simulink model "stall_detection_block_v2"  (R2022b)
settings: Solver=FixedStepAuto  StartTime=0.0  StopTime=inf  FixedStep=0.002  RelTol=1e-3  EnableMultiTasking=on
undefined symbols (not defined in the file or in its folder): DiscIntNeverNeededParam
libraries: quarc_library x1
settings Model: Creator=christopher.oneill  LastModifiedBy=christopher.oneill
settings SolverCC: PositivePriorityOrder=on
settings RTWCC: Description=QUARC Win64 Target Using Toolchain  SystemTargetFile=quarc_win64.tlc  Toolchain=QUARC win64 | nmake (64-bit Windows)  BuildConfiguration=Faster Runs
settings STFCustomTargetCC: TargetLangStandard=C99 (ISO)  ConcurrentExecutionCompliant=on  GRTInterface=on  UseToolchainInfoCompliant=on  SystemTargetFile=quarc_win64.tlc
settings GRTTargetCC: ParMdlRefBuildCompliant=off  CompOptLevelCompliant=off  CombineOutputUpdateFcns=off  MatFileLogging=off  CPPClassGenCompliant=off  GRTInterface=on  ExtMode=on  ExtModeMexFile=quarc_comm

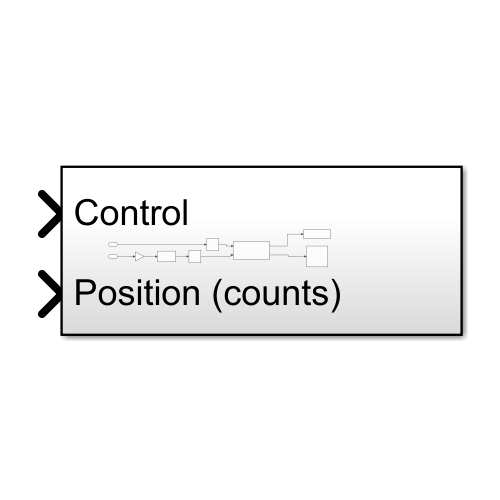
[thumbnail: Simulink's stored preview of the top-level diagram]
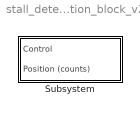
== system stall_detection_block_v2 ==
  Subsystem : Subsystem

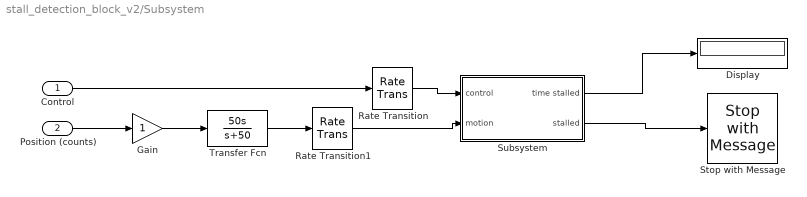
== system stall_detection_block_v2/Subsystem ==
  Control : Inport
  Position (counts) : Inport  Port=2
  Display : Display
  Gain : Gain
  Rate Transition : RateTransition
  Rate Transition1 : RateTransition
  Stop with Message : quarc_library/Sinks/Error Handling/Stop with Message  message_type=Fixed error message  message_icon=Error  message=Stall Detected! Please snsure that the DC motor is free to move and is functioning properly. Please ask a TA to check your code if you have recived this error.
  Subsystem : Subsystem
  Transfer Fcn : TransferFcn  Numerator=[50 0]  Denominator=[1 50]
  wires:
  Control/1 -> Rate Transition/1
  Position (counts)/1 -> Gain/1
  Gain/1 -> Transfer Fcn/1
  Transfer Fcn/1 -> Rate Transition1/1
  Rate Transition1/1 -> Subsystem/2(motion)
  Rate Transition/1 -> Subsystem/1(control)
  Subsystem/1(time stalled) -> Display/1
  Subsystem/2(stalled) -> Stop with Message/1

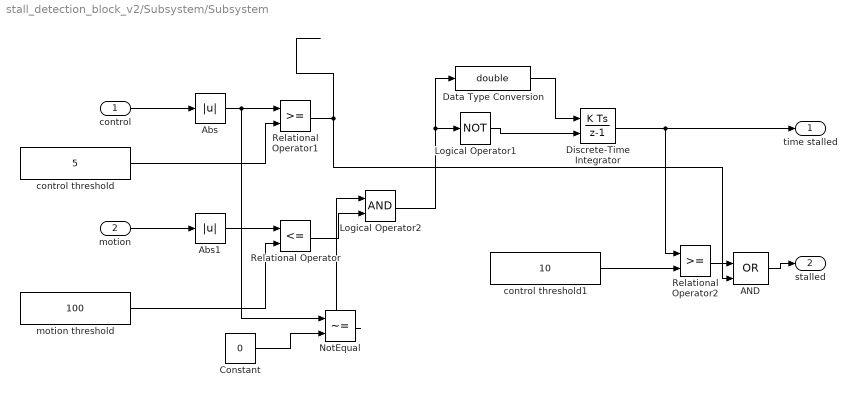
== system stall_detection_block_v2/Subsystem/Subsystem ==
  control : Inport
  motion : Inport  Port=2
  AND : Logic  Operator=OR  IconShape=distinctive  AllPortsSameDT=off  OutDataTypeStr=boolean
  Abs : Abs  SaturateOnIntegerOverflow=off
  Abs1 : Abs  SaturateOnIntegerOverflow=off
  Constant : Constant  Value=0
  Data Type Conversion : DataTypeConversion  OutDataTypeStr=double  SaturateOnIntegerOverflow=off  RndMeth=Floor
  Discrete-Time Integrator : DiscreteIntegrator  ExternalReset=rising  InitialConditionSetting=Compatibility  SampleTime=-1  ICPrevOutput=DiscIntNeverNeededParam  ICPrevScaledInput=DiscIntNeverNeededParam
  Logical Operator1 : Logic  Operator=NOT  AllPortsSameDT=off  OutDataTypeStr=boolean
  Logical Operator2 : Logic  AllPortsSameDT=off  OutDataTypeStr=boolean
  NotEqual : RelationalOperator  Operator=~=  OutDataTypeStr=boolean  RndMeth=Simplest  InputSameDT=off
  Relational Operator : RelationalOperator  Operator=<=  OutDataTypeStr=boolean  InputSameDT=off
  Relational Operator1 : RelationalOperator  OutDataTypeStr=boolean  InputSameDT=off
  Relational Operator2 : RelationalOperator  OutDataTypeStr=boolean  InputSameDT=off
  control threshold : Constant  Value=5
  control threshold1 : Constant  Value=10
  motion threshold : Constant  Value=100
  time stalled : Outport
  stalled : Outport  Port=2
  wires:
  motion/1 -> Abs1/1
  Logical Operator2/1 -> Logical Operator1/1, Data Type Conversion/1
  motion threshold/1 -> Relational Operator/2
  control threshold/1 -> Relational Operator1/2
  Abs/1 -> NotEqual/1, Relational Operator1/1
  control/1 -> Abs/1
  Logical Operator1/1 -> Discrete-Time Integrator/2
  Discrete-Time Integrator/1 -> time stalled/1, Relational Operator2/1
  Data Type Conversion/1 -> Discrete-Time Integrator/1
  Abs1/1 -> Relational Operator/1
  control threshold1/1 -> Relational Operator2/2
  Constant/1 -> NotEqual/2
  Relational Operator1/1 -> AND/2
  Relational Operator2/1 -> AND/1
  AND/1 -> stalled/1
  Relational Operator/1 -> Logical Operator2/2
  NotEqual/1 -> Logical Operator2/1
